simulink model "PV_SYSTEM_WITH_VARIOUS_MPPT"  (R2017a)
settings: Solver=ode45  StartTime=0.0  StopTime=2  RelTol=1e-3  EnableMultiTasking=on
undefined symbols (not defined in the file): dEgdT, EgRef, gcbh, k1, Rsh_array5pc, sigbuilder_block, sps_rtmsupport, Tref_K, Ts, VT_ref
libraries: powerlib x16, neural x15, simulink x4, spsPVarrayModel x3, powerlib_extras x2, fuzblock x1, powerlib_meascontrol x1
(part 1 of 6)
settings Model: Creator=Sanjay Lodwal  LastModifiedBy=seybo
settings DataIOCC: LimitDataPoints=on  SaveFormat=Array
settings OptimizationCC: LifeSpan=inf
settings DebuggingCC: UnderspecifiedInitializationDetection=Classic  MergeDetectMultiDrivingBlocksExec=none  MaxConsecutiveZCsMsg=none  SolverPrmCheckMsg=warning  StateNameClashWarn=warning  SFUnexpectedBacktrackingDiag=warning  SFNoUnconditionalDefaultTransitionDiag=warning  SFExecutionAtInitializationDiag=none
settings HardwareCC: ProdBitPerPointer=32  ProdBitPerSizeT=32  ProdBitPerPtrDiffT=32  ProdLargestAtomicFloat=None  ProdIntDivRoundTo=Undefined  ProdEndianess=Unspecified  ProdWordSize=32  ProdHWDeviceType=32-bit Generic
settings ModelReferenceCC: PropagateSignalLabelsOutOfModel=off
settings GRTTargetCC: TargetLangStandard=C89/C90 (ANSI)  GeneratePreprocessorConditionals=Disable all
settings ConfigComp: CovMetricSettings=dw  CovHtmlReporting=on  CovSaveCumulativeToWorkspaceVar=on  CovSaveSingleToWorkspaceVar=on  CovExternalEMLEnable=off

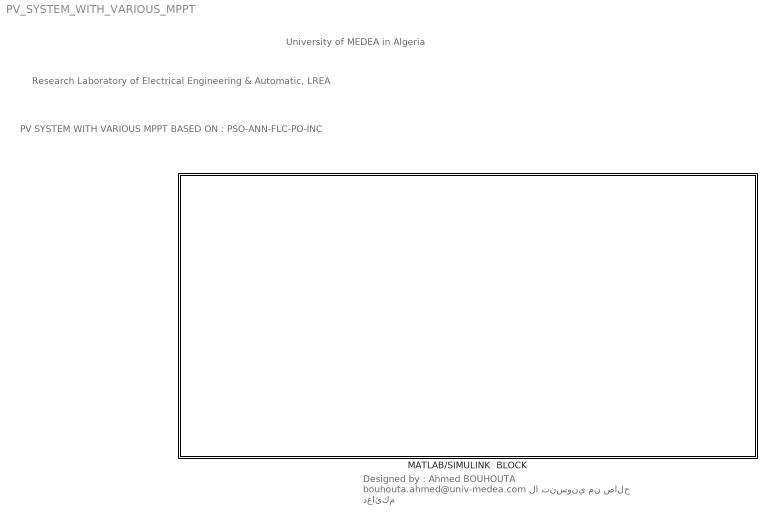
== system PV_SYSTEM_WITH_VARIOUS_MPPT ==
  note: University of MEDEA in Algeria
  note: Research Laboratory of Electrical Engineering & Automatic, LREA
  note: Designed by : Ahmed BOUHOUTA
      | bouhouta.ahmed@univ-medea.com
      | لا تنسوني من صالح دعائكم
  note: PV SYSTEM WITH VARIOUS MPPT BASED ON : PSO-ANN-FLC-PO-INC
  MATLAB/SIMULINK  BLOCK : Subsystem
      mask Display: image(imread('MPPT.jpg'))

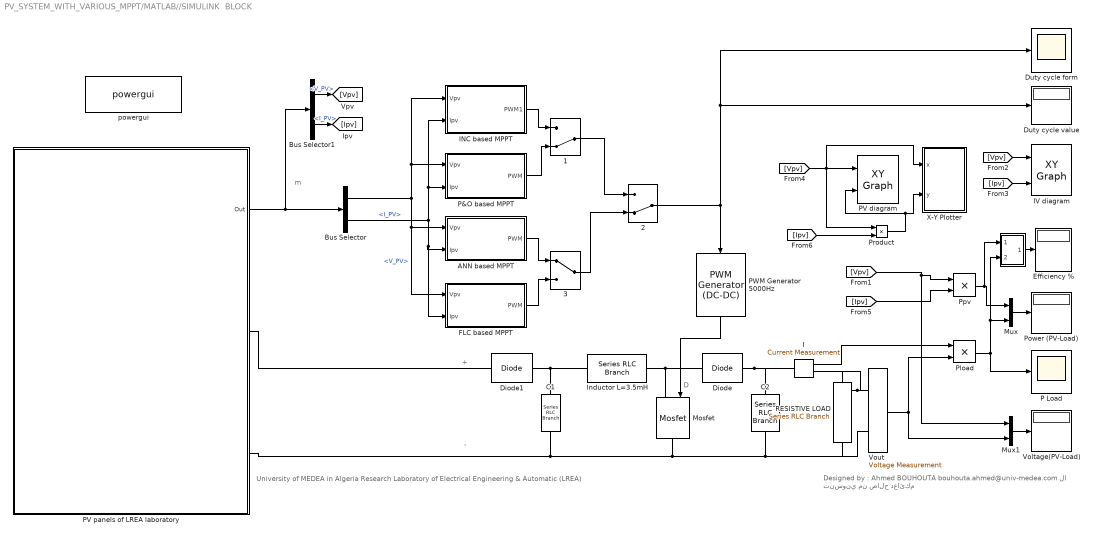
== system PV_SYSTEM_WITH_VARIOUS_MPPT/MATLAB//SIMULINK  BLOCK ==
  note: -
  note: D
  note: m
  note: +
  note: University of MEDEA in Algeria
      | Research Laboratory of Electrical Engineering & Automatic (LREA)
  note: Designed by : Ahmed BOUHOUTA
      | bouhouta.ahmed@univ-medea.com
      | لا تنسوني من صالح دعائكم
  "\tPV panels of LREA laboratory " : Subsystem
      mask Display: image(imread('imagePV1.jpg'))
  "     " : Subsystem
  "      1" : ManualSwitch  CurrentSetting=0
  "      2" : ManualSwitch  CurrentSetting=0
  "      3" : ManualSwitch
  ANN based MPPT : Subsystem
  Bus Selector : BusSelector  OutputSignals=V_PV,I_PV
  Bus Selector1 : BusSelector  OutputSignals=V_PV,I_PV
  C1 : powerlib/Elements/Series RLC Branch  LConnTagsString=__new0  RConnTagsString=__new0  BranchType=C  Resistance=0.001  Inductance=1.0  SetiL0=off  InitialCurrent=0  Capacitance=200e-6  Setx0=off  InitialVoltage=310  Measurements=None
  C2 : powerlib/Elements/Series RLC Branch  LConnTagsString=__new0  RConnTagsString=__new0  BranchType=C  Resistance=1  Inductance=1e-3  SetiL0=off  InitialCurrent=0  Capacitance=100e-6  Setx0=off  InitialVoltage=600  Measurements=None
  Diode : powerlib/Power Electronics/Diode  Ron=0.001  Lon=0  Vf=0.8  IC=0  UseSnubber=off  Rs=500  Cs=250e-9  Measurements=off
  Diode1 : powerlib/Power Electronics/Diode  Ron=0.001  Lon=0  Vf=0.8  IC=0  UseSnubber=off  Rs=500  Cs=250e-9  Measurements=off
  Duty cycle form : Scope
  Duty cycle value : Display
  Efficiency % : Display
  FLC based MPPT : Subsystem
  I : powerlib/Measurements/Current Measurement  PhasorSimulation=off  OutputType=Complex  PSBequivalent=0
  INC based MPPT : Subsystem
  IV diagram : simulink/Sinks/XY Graph  xmin=0  xmax=110  ymin=0  ymax=5  st=0.0001
  Inductor L=3.5mH : powerlib/Elements/Series RLC Branch  LConnTagsString=__new0  RConnTagsString=__new0  BranchType=L  Resistance=0.01  Inductance=3.5e-3  SetiL0=on  InitialCurrent=5  Capacitance=1e-6  Setx0=off  InitialVoltage=0  Measurements=None
  Mosfet : powerlib/Power Electronics/Mosfet  Ron=0.1  Lon=0  Rd=0.01  Vfd=0  IC=0  Rs=1e5  Cs=inf  Measurements=off
  Mux : Mux  Inputs=2
  Mux1 : Mux  Inputs=2
  P Load : Scope
  P&O based MPPT : Subsystem
  PV diagram : simulink/Sinks/XY Graph  xmin=0  xmax=210  ymin=0  ymax=450  st=0.0001
  "PWM Generator 5000Hz " : powerlib_meascontrol/Pulse & Signal Generators/PWM Generator (DC-DC)  Fsw=5000  Ts=1e-6
  Pload : Product
  Power (PV-Load) : Display
  Ppv : Product
  Product : Product
  RESISTIVE LOAD : powerlib/Elements/Series RLC Branch  LConnTagsString=__new0  RConnTagsString=__new0  BranchType=R  Resistance=300  Inductance=1e-3  SetiL0=off  InitialCurrent=0  Capacitance=1e-6  Setx0=off  InitialVoltage=0  Measurements=None
  Voltage(PV-Load) : Display
  Vout : powerlib/Measurements/Voltage Measurement  PhasorSimulation=off  OutputType=Complex  PSBequivalent=0
  X-Y Plotter : Subsystem  mask{N=50, tsam=1e-6, xmin=0, xmax=200, ymin=0, ymax=450}
      mask prompts: N "Number of Sample, N"; tsam "Sample Time, tsam (s)"; xmin "Minimum Limit of X, xmin"; xmax "Maximum Limit of X, xmin"; ymin "Minimum Limit of Y, ymin"; ymax "Maximum Limit of Y, ymin"
      mask DialogControl DescGroupVar Prompt: X-Y Plotter
      mask DialogControl DescTextVar Prompt: X-Y Animated Plotter with Reference
      mask DialogControl Control2 Prompt: N <=10,000. If N>10,000, change mem inside the function.
      mask DialogControl Control3 Prompt: Razman Ayop
      mask DialogControl Control7 Prompt: Homepage
      mask DialogControl Control7 Callback: web('https://people.utm.my/razman-ayop/')
      mask DialogControl Control4 Prompt: Created on 7 Nov 19
      mask Display: plot([.05 .95 .95 .05 .05],[.45 .45 .95 .95 .45], 0.5+cos(0:0.1:2*pi)*0.3,0.7+sin(0:0.1:2*pi)*0.2)
  powergui : powerlib/powergui  Priority=1  SimulationMode=Discrete  SampleTime=1e-6  frequency=60  Iterations=50  frequencyindice=0  Pbase=100e6  ErrMax=1e-4  UnitsV=kV  UnitsW=MW  buscounter=0  FunctionMessages=off  echomessages=off  EnableUseOfTLC=off  CurrentSourceSwitches=off  DisableSnubberDevices=off  DisableRonSwitches=off  DisableVfSwitches=off  DisplayEquations=off  SolverType=Tustin/Backward Euler (TBE)  Interpol=off  ExternalGateDelay=off  methode=off  Ts=100  x0status=blocks  SPID=off  SwTol=0  HookPort=off  RestoreLinks=warning  ResistiveCurrentMeasurement=off  Frange=[0:2:500]  Ylog=off  Xlog=on  ShowGrid=off  save=off  variable=ZData  structure=0  ZoomFFT=off  StartTime=0.0  cycles=1  DisplayStyle=1  fundamental=60  FreqAxis=off  MaxFrequency=1000  frequencyindicesteady=1  RmsSteady=1  display=off
  wires:
  Bus Selector1/1 -> [Vpv]  "<V_PV>"
  [Vpv] -> Mux1/1, Ppv/1
  Mux/1 -> Power (PV-Load)/1
  "\tPV panels of LREA laboratory "/1(Out) -> Bus Selector1/1, Bus Selector/1
  "      3"/1 -> "      2"/2
  INC based MPPT/1(PWM1) -> "      1"/1
  "      1"/1 -> "      2"/1
  Bus Selector/1 -> INC based MPPT/1(Vpv), P&O based MPPT/1(Vpv), FLC based MPPT/1(Vpv), ANN based MPPT/1(Vpv)  "<V_PV>"
  [Ipv] -> Ppv/2
  [Ipv] -> IV diagram/2
  [Vpv] -> IV diagram/1
  P&O based MPPT/1(PWM) -> "      1"/2
  Pload/1 -> P Load/1, "     "/2(In2), Mux/2
  Bus Selector/2 -> INC based MPPT/2(Ipv), P&O based MPPT/2(Ipv), FLC based MPPT/2(Ipv), ANN based MPPT/2(Ipv)  "<I_PV>"
  ANN based MPPT/1(PWM) -> "      3"/1
  Mux1/1 -> Voltage(PV-Load)/1
  Bus Selector1/2 -> [Ipv]  "<I_PV>"
  I/1 -> Pload/1
  FLC based MPPT/1(PWM) -> "      3"/2
  Ppv/1 -> "     "/1(In1), Mux/1
  "PWM Generator 5000Hz "/1 -> Mosfet/1
  Vout/1 -> Pload/2, Mux1/2
  "     "/1(Out1) -> Efficiency %/1
  "      2"/1 -> Duty cycle form/1, Duty cycle value/1, "PWM Generator 5000Hz "/1
  [Vpv] -> X-Y Plotter/1(x), Product/1, PV diagram/1
  Product/1 -> PV diagram/2, X-Y Plotter/2(y)
  [Ipv] -> Product/2
  connections:
  Mosfet/LConn1 -- Diode/LConn1 -- Inductor L=3.5mH/RConn1
  Vout/LConn1 -- I/RConn1 -- RESISTIVE LOAD/LConn1
  Diode/RConn1 -- C2/LConn1 -- I/LConn1
  RESISTIVE LOAD/RConn1 -- Vout/LConn2 -- C2/RConn1 -- Mosfet/RConn1 -- "\tPV panels of LREA laboratory "/RConn2 -- C1/RConn1
  Diode1/RConn1 -- Inductor L=3.5mH/LConn1 -- C1/LConn1
  Diode1/LConn1 -- "\tPV panels of LREA laboratory "/RConn1
